simulink model "stardelta"  (R2024b)
settings: Solver=ode23tb  StartTime=0.0  StopTime=3  MaxStep=1e-4  RelTol=1e-3
undefined symbols (not defined in the file or in its folder): D1, Delta
libraries: spsThreePhaseVIMeasurementLib x3, spsThreePhaseBreakerLib x3, spsThreePhaseTransformerTwoWindingsLib x2, spsAsynchronousMachineSIUnitsLib x1, spsCurrentMeasurementLib x1, spsRMSLib x1, spsThreePhaseSeriesRLCLoadLib x1, spsThreePhaseSourceLib x1, spsVoltageMeasurementLib x1, sps_lib x1
settings Model: PacingRate=112  Creator=aminbgr  LastModifiedBy=aminbgr

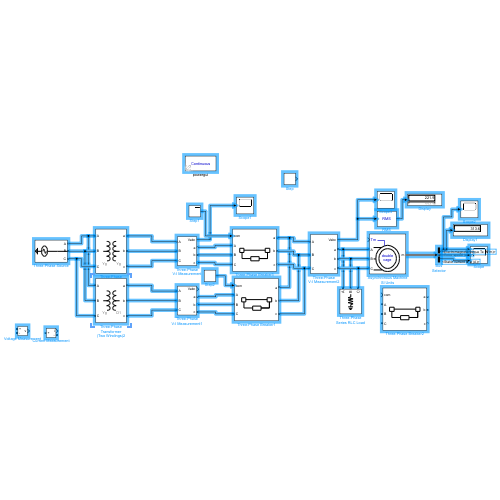
[thumbnail: Simulink's stored preview of the top-level diagram]
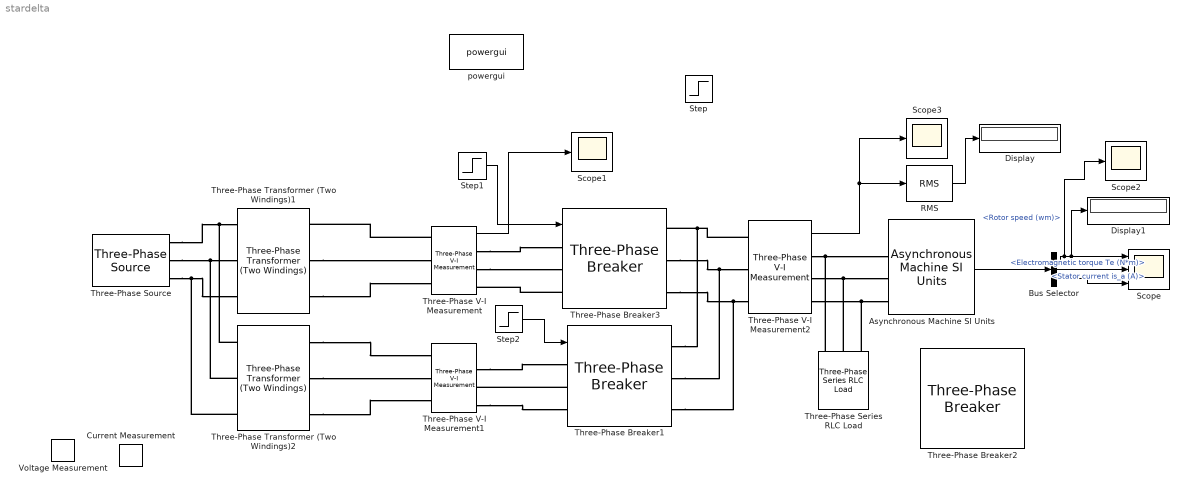
== system stardelta ==
  Asynchronous Machine SI Units : spsAsynchronousMachineSIUnitsLib/Asynchronous Machine SI Units  RotorType=Double squirrel-cage  PresetModel=No  MechanicalLoad=Torque Tm  ShowDetailedParameters=on  ReferenceFrame=Rotor  Units=SI  MeasurementBus=off  NominalParameters=[9.007e+04 400 50]  VoltageRatio=1  Stator=[0.05751 0.0001929]  Rotor=[0.6258 0.005473]  Cage1=[0.01311 0.0005295]  Cage2=[0.305 0.0001929]  Lm=0.01395  Mechanical=[0.94 0.005879 1]  PolePairs=2  InitialConditions=[1 0 0 0 0 0 0 0]  SimulateSaturation=off  Saturation=[14.03593122, 27.81365428, 53.79336849, 72.68890987, 97.98006896, 148.6815601, 215.7428561, 302.9841135, 428.7778367 ; 230, 322, 414, 460, 506, 552, 598, 644, 690]  LoadFlowParameters=1492000  TsPowergui=0  TsBlock=-1  IterativeModel=Trapezoidal non iterative  IterativeDiscreteModel=Trapezoidal non iterative  Pmec=0
  Bus Selector : BusSelector  OutputSignals=Mechanical.Rotor speed (wm),Mechanical.Electromagnetic torque Te (N*m),Stator measurements.Stator current is_a (A)
  Current Measurement : spsCurrentMeasurementLib/Current Measurement  PhasorSimulation=off  OutputType=Complex  PSBequivalent=0
  Display : Display
  Display1 : Display
  RMS : spsRMSLib/RMS  TrueRMS=on  Freq=60  RMSInit=120  Ts=0
  Scope : Scope  NumInputPorts=3
  Scope1 : Scope
  Scope2 : Scope
  Scope3 : Scope
  Step : Step  Time=0.5  SampleTime=0
  Step1 : Step  SampleTime=0
  Step2 : Step  Time=6  SampleTime=0
  Three-Phase Series RLC Load : spsThreePhaseSeriesRLCLoadLib/Three-Phase Series RLC Load  LConnTagsString=A|B|C  Configuration=Y (grounded)  NominalVoltage=400  Vabc=[1e3 1e3 1e3]  Vabcp=[1e3 1e3 1e3]  NominalFrequency=50  UnbalancedPower=off  ActivePower=10  InductivePower=0  CapacitivePower=0  Pabc=[10e3 9e3 11e3]  QLabc=[100 90 110]  QCabc=[100 90 110]  Pabcp=[10e3 9e3 11e3]  QLabcp=[100 90 110]  QCabcp=[100 90 110]  Measurements=None  LoadType=constant Z
  Three-Phase Transformer (Two Windings)1 : spsThreePhaseTransformerTwoWindingsLib/Three-Phase Transformer (Two Windings)  Winding1Connection=Yg  Winding2Connection=Yg  CoreType=Three single-phase transformers  SetSaturation=off  Hysteresis=off  DataFile='hysteresis'  SetInitialFlux=off  Measurements=Winding voltages  UNITS=pu  NominalPower=[ 125e3 50 ]  Winding1=[20e3 0.005 0.02]  Winding2=[400/sqrt(3) 0.005 0.02]  Rm=500  Lm=500  L0=0.004  Saturation=[0 0;0.075409 63.654;31.42 80.627]  InitialFluxes=[42.436 -42.436 37.132]  BreakLoop=off  DiscreteSolver=Trapezoidal iterative  DataType=off  TransfoNumber=1
  Three-Phase Transformer (Two Windings)2 : spsThreePhaseTransformerTwoWindingsLib/Three-Phase Transformer (Two Windings)  Winding1Connection=Yg  Winding2Connection=Delta (D1)  CoreType=Three single-phase transformers  SetSaturation=off  Hysteresis=off  DataFile='hysteresis'  SetInitialFlux=off  Measurements=Winding voltages  UNITS=pu  NominalPower=[ 125e3 50 ]  Winding1=[20e3 0.005 0.02]  Winding2=[400 0.005 0.02]  Rm=500  Lm=500  L0=0.004  Saturation=[0 0;0.075409 63.654;31.42 80.627]  InitialFluxes=[42.436 -42.436 37.132]  BreakLoop=off  DiscreteSolver=Trapezoidal iterative  DataType=off  TransfoNumber=1
  Three-Phase V-I Measurement : spsThreePhaseVIMeasurementLib/Three-Phase V-I Measurement  VoltageMeasurement=phase-to-phase  SetLabelV=off  LabelV=Vabc  Vpu=off  VpuLL=off  CurrentMeasurement=no  SetLabelI=off  LabelI=Iabc  Ipu=off  Pbase=100e6  Vbase=500e3  OutputType=Complex  PhasorSimulation=off  PSBequivalent=0
  Three-Phase V-I Measurement1 : spsThreePhaseVIMeasurementLib/Three-Phase V-I Measurement  VoltageMeasurement=phase-to-phase  SetLabelV=off  LabelV=Vabc  Vpu=off  VpuLL=off  CurrentMeasurement=no  SetLabelI=off  LabelI=Iabc  Ipu=off  Pbase=100e6  Vbase=500e3  OutputType=Complex  PhasorSimulation=off  PSBequivalent=0
  Three-Phase V-I Measurement2 : spsThreePhaseVIMeasurementLib/Three-Phase V-I Measurement  VoltageMeasurement=phase-to-phase  SetLabelV=off  LabelV=Vabc  Vpu=off  VpuLL=off  CurrentMeasurement=no  SetLabelI=off  LabelI=Iabc  Ipu=off  Pbase=100e6  Vbase=500e3  OutputType=Complex  PhasorSimulation=off  PSBequivalent=0
  Three-Phase Breaker1 : spsThreePhaseBreakerLib/Three-Phase Breaker  InitialState=closed  SwitchA=on  SwitchB=on  SwitchC=on  SwitchTimes="[1/60  5/60]"  External=on  BreakerResistance=0.01  SnubberResistance=1e6  SnubberCapacitance=inf  Measurements=None
  Three-Phase Breaker2 : spsThreePhaseBreakerLib/Three-Phase Breaker  InitialState=closed  SwitchA=on  SwitchB=on  SwitchC=on  SwitchTimes="[1/60  5/60]"  External=on  BreakerResistance=0.01  SnubberResistance=1e6  SnubberCapacitance=inf  Measurements=None
  Three-Phase Breaker3 : spsThreePhaseBreakerLib/Three-Phase Breaker  InitialState=closed  SwitchA=on  SwitchB=on  SwitchC=on  SwitchTimes="[1/60  5/60]"  External=on  BreakerResistance=0.01  SnubberResistance=1e6  SnubberCapacitance=inf  Measurements=None
  Three-Phase Source : spsThreePhaseSourceLib/Three-Phase Source  InternalConnection=Yg  VoltagePhases=off  Voltage=20e+3  PhaseAngle=0  Voltage_phases=[25e3 25e3 25e3]/sqrt(3)  PhaseAngles_phases=[0 -120 +120]  Frequency=50  NonIdealSource=off  SpecifyImpedance=off  Resistance=0.8929  Inductance=16.58e-3  ShortCircuitLevel=100e6  BaseVoltage=25e3  XRratio=7  BusType=swing  Pref=10e3  Qref=0  Prefabc=[10e3, 10e3, 10e3]  Qrefabc=[0, 0, 0]  Qmin=-inf  Qmax=inf
  Voltage Measurement : spsVoltageMeasurementLib/Voltage Measurement  PhasorSimulation=off  OutputType=Complex  PSBequivalent=0
  powergui : sps_lib/powergui  Priority=1  SimulationMode=Continuous  SampleTime=50e-6  frequency=60  Iterations=50  frequencyindice=50  Pbase=100e6  ErrMax=1e-4  UnitsV=kV  UnitsW=MW  buscounter=0  FunctionMessages=off  echomessages=off  EnableUseOfTLC=off  CurrentSourceSwitches=off  DisableSnubberDevices=off  DisableRonSwitches=off  DisableVfSwitches=off  DisplayEquations=off  AutomaticDiscreteSolvers=off  SolverType=Tustin/Backward Euler (TBE)  Interpol=off  ExternalGateDelay=off  methode=off  Ts=100  x0status=blocks  SPID=on  SwTol=0  HookPort=off  NonlinearTolerance=1e-4  nMaxIteration=100  ContinueOnMaxIteration=off  RestoreLinks=warning  ResistiveCurrentMeasurement=off  Frange=[0:2:500]  Ylog=off  Xlog=on  ShowGrid=off  save=off  variable=ZData  structure=0  ZoomFFT=off  StartTime=0.0  cycles=1  DisplayStyle=1  fundamental=60  FreqAxis=off  MaxFrequency=1000  frequencyindicesteady=1  RmsSteady=1  display=off
  wires:
  Asynchronous Machine SI Units/1 -> Bus Selector/1
  Bus Selector/1 -> Scope2/1, Display1/1, Scope/1  "<Rotor speed (wm)>"
  Bus Selector/2 -> Scope/2  "<Electromagnetic torque Te (N*m)>"
  Bus Selector/3 -> Scope/3  "<Stator current is_a (A)>"
  RMS/1 -> Display/1
  Three-Phase V-I Measurement2/1 -> Scope3/1, RMS/1
  Three-Phase V-I Measurement/1 -> Scope1/1
  Step2/1 -> Three-Phase Breaker1/1
  Step1/1 -> Three-Phase Breaker3/1
  connections:
  Three-Phase V-I Measurement2/RConn1 -- Three-Phase Series RLC Load/LConn1 -- Asynchronous Machine SI Units/LConn1
  Three-Phase V-I Measurement2/RConn2 -- Three-Phase Series RLC Load/LConn2 -- Asynchronous Machine SI Units/LConn2
  Three-Phase V-I Measurement2/RConn3 -- Three-Phase Series RLC Load/LConn3 -- Asynchronous Machine SI Units/LConn3
  Three-Phase Source/RConn1 -- Three-Phase Transformer (Two Windings)2/LConn1 -- Three-Phase Transformer (Two Windings)1/LConn1
  Three-Phase Source/RConn2 -- Three-Phase Transformer (Two Windings)2/LConn2 -- Three-Phase Transformer (Two Windings)1/LConn2
  Three-Phase Source/RConn3 -- Three-Phase Transformer (Two Windings)2/LConn3 -- Three-Phase Transformer (Two Windings)1/LConn3
  Three-Phase V-I Measurement/LConn1 -- Three-Phase Transformer (Two Windings)1/RConn1
  Three-Phase Transformer (Two Windings)1/RConn2 -- Three-Phase V-I Measurement/LConn2
  Three-Phase Transformer (Two Windings)1/RConn3 -- Three-Phase V-I Measurement/LConn3
  Three-Phase Transformer (Two Windings)2/RConn1 -- Three-Phase V-I Measurement1/LConn1
  Three-Phase Transformer (Two Windings)2/RConn2 -- Three-Phase V-I Measurement1/LConn2
  Three-Phase Transformer (Two Windings)2/RConn3 -- Three-Phase V-I Measurement1/LConn3
  Three-Phase V-I Measurement1/RConn1 -- Three-Phase Breaker1/LConn1
  Three-Phase Breaker1/LConn2 -- Three-Phase V-I Measurement1/RConn2
  Three-Phase V-I Measurement1/RConn3 -- Three-Phase Breaker1/LConn3
  Three-Phase V-I Measurement/RConn1 -- Three-Phase Breaker3/LConn1
  Three-Phase V-I Measurement/RConn2 -- Three-Phase Breaker3/LConn2
  Three-Phase Breaker3/LConn3 -- Three-Phase V-I Measurement/RConn3
  Three-Phase V-I Measurement2/LConn1 -- Three-Phase Breaker1/RConn1 -- Three-Phase Breaker3/RConn1
  Three-Phase Breaker3/RConn2 -- Three-Phase Breaker1/RConn2 -- Three-Phase V-I Measurement2/LConn2
  Three-Phase Breaker3/RConn3 -- Three-Phase Breaker1/RConn3 -- Three-Phase V-I Measurement2/LConn3
